simulink model "PID20ejeYanalnivels"  (Simulink 6.6)
settings: Solver=FixedStepDiscrete  StartTime=0.0  StopTime=.002  FixedStep=0.001  RelTol=1e-3
libraries: dsPICdrivers x10, simulink x3
settings Model: Creator=123  LastModifiedBy=123  ProdHWDeviceType=16-bit Generic
settings OptimizationCC: OptimizeModelRefInitCode=on  LifeSpan=1
settings HardwareCC: ProdBitPerInt=16  ProdEndianess=LittleEndian  ProdWordSize=16  ProdHWDeviceType=16-bit Generic  TargetHWDeviceType=32-bit Generic
settings RTWCC: SystemTargetFile=dspic.tlc  TemplateMakefile=dspic_pic30_gcc.tmf  PostCodeGenCommand=dsPIC_Compile()  Description=Embedded Target for Microchip dsPIC (real-time)  ProcessScript=dspic_make_rtw_hook  CustomSource=myQEI.c
settings CodeAppCC: IgnoreCustomStorageClasses=off
settings STFCustomTargetCC: TargetFcnLib=ansi_tfl_tmw.mat  GenFloatMathFcnCalls=ANSI_C  ModelReferenceCompliant=off  IncludeMdlTerminateFcn=off  CombineOutputUpdateFcns=on  SuppressErrorStatus=on  ERTCustomFileBanners=on  SupportContinuousTime=off  SupportNonInlinedSFcns=off  SystemTargetFile=dspic.tlc
settings ERTTargetCC: TargetFcnLib=ansi_tfl_tmw.mat  GenFloatMathFcnCalls=ANSI_C  ModelReferenceCompliant=off  IncludeMdlTerminateFcn=off  SuppressErrorStatus=on  ModelStepFunctionPrototypeControlCompliant=off  InlinedParameterPlacement=NonHierarchical  ERTSrcFileBannerTemplate=dsPIC_code_template.cgt  ERTHdrFileBannerTemplate=dsPIC_code_template.cgt  ERTDataSrcFileTemplate=dsPIC_code_template.cgt  ERTDataHdrFileTemplate=dsPIC_code_template.cgt  ERTCustomFileTemplate=dsPIC_main.tlc
settings CustomProperty: DataType=string  Value=C:\PROGRA~2\MATLAB\R2007a\rtw\bin\win32\gmake

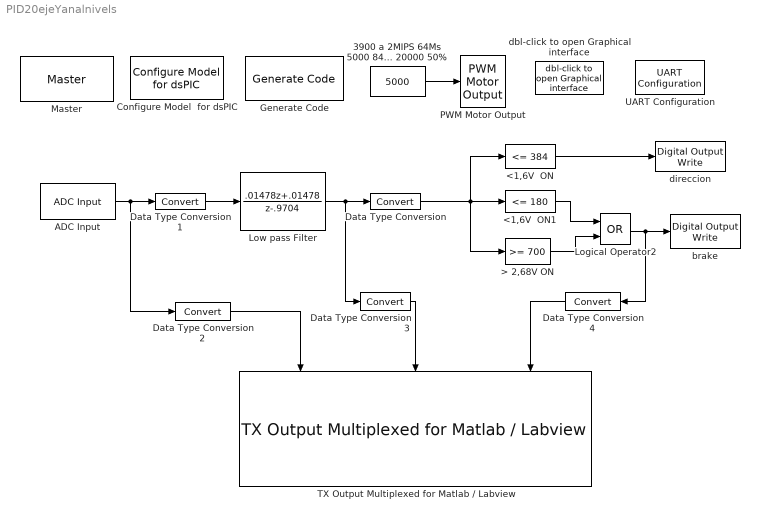
== system PID20ejeYanalnivels ==
  3900 a 2MIPS 64Ms 5000 84Ms 40000 full 20000 50% : Constant  Value=5000  OutDataTypeMode=uint16  SampleTime=.001
  <1,6V  ON : simulink/Logic and Bit Operations/Compare To Constant  SystemSampleTime=-1  relop=<=  const=384  LogicOutDataTypeMode=boolean  ZeroCross=off
  <1,6V  ON1 : simulink/Logic and Bit Operations/Compare To Constant  SystemSampleTime=-1  relop=<=  const=180  LogicOutDataTypeMode=boolean  ZeroCross=off
  > 2,68V ON : simulink/Logic and Bit Operations/Compare To Constant  SystemSampleTime=-1  relop=>=  const=700  LogicOutDataTypeMode=boolean  ZeroCross=off
  ADC Input : dsPICdrivers/Peripheral I//O/ADC Input  Tag=dsPIC_ADC  Priority=5  ADC_TYPE=10 bits  ADC_MODE=Continuous sampling & get last channel value  NbrSampleStep=1  VoltRefpopup="AVdd  -  AVss"  OutFormatBitspopup=0000 00dd dddd dddd : Integer  InterruptPriority=1  ANCHANNELS=[0]  MaxName=ANmax = 1024  Rin=1e2  ADCS=9  SAMC=1  Temperature=25  DMAChannel=0  SampleTime=.001  Status="OK  |  Tsmp=1.667e-007 |  T/Channel=2.167e-006 |  Tall=2.167e-006"
  Configure Model  for dsPIC : dsPICdrivers/Simulink Configuration/Configure Model  for dsPIC
  Data Type Conversion : DataTypeConversion  OutDataTypeMode=uint16  SampleTime=.001
  Data Type Conversion1 : DataTypeConversion  OutDataTypeMode=double  SampleTime=.001
  Data Type Conversion2 : DataTypeConversion  OutDataTypeMode=int16  SampleTime=.001
  Data Type Conversion3 : DataTypeConversion  OutDataTypeMode=int16  SampleTime=.001
  Data Type Conversion4 : DataTypeConversion  Orientation=left  OutDataTypeMode=int16  SampleTime=.001
  Generate Code : dsPICdrivers/Simulink Configuration/Generate Code
  Logical Operator2 : Logic  Operator=OR  AllPortsSameDT=off  OutDataTypeMode=Boolean  SampleTime=.001
  Low pass Filter : DiscreteTransferFcn  Numerator="[.01478  .01478]"  Denominator=[1 -.9704]  SampleTime=.001
  Master : dsPICdrivers/Master  Tag=dsPIC_MASTER  Priority=1  TimeStepType=Timer1  picType=30f4012  fcy=30e6  Quartz_33f=5e6  PLLActive_33f=off  fcyDesired_33f=0  tmr1="[1  29999  0]"  tmr1Info="Time Step : 0.001  ;   Error : 0%  PR1=29999"  tmr2345="[0  0  0  0]"  tmr2345cfg=[-1 -1 -1 -1]  IOautoConf=on  typePort="[ 0   0   0   0   0   0   0   0   0   0   0   0   0   0   0   0   8   0   0   0   0   0   0   0   0   0   0   0   0   0   0   0   0   0   0   0   0   0   0   0   0   0   0   0   0   0   0   0  10  10   0   0   0   0   0   0   0   0   0   0   0   0   0   0  11   0   0   0   0   0   0   0   0   0   0   0   0   0   0   0   0   0   4   5   0   0   0   0   0   0   0   0   0   0   0   0   0   0   0   0   0   0   0   0   0   0   0   0   0   0   0   0 ]"  TRIS="[ 65535  65535  65535  65532  65535  65535  65535 ]"  ADPCFG=0  MasterBusyPort=None  MasterOverloadPort=None  FOSC=FRC_PLL16  ClockSwitchMonitor=Both disabled  TempProtection_33f=TEMP_ON  FPBOR=PBOR_OFF  PWRT=PWRT_OFF  MCLR=MCLR_DIS  PowerSave=off  OverrideFcy=off  NewFcy=1e6
  PWM Motor Output : dsPICdrivers/Peripheral I//O/PWM Motor Output  Tag=dsPIC_PWM_Motor  Priority=5  InputEnableChk=off  InputPeriodeChk=off  Channel=[1 ]  TPeriode=.01  PrescalerValue=16  PeriodeInteger=18750  MaxName='PWM'  Centered=off  HChannelON=off  Info="Nbr Bits : 15.1946  ||  PWM = 37500  ||  Prescaler = 16"  Delay=0  IntPriority=5  nbrPwmChannelPIC=3  Status=OK
  TX Output Multiplexed for Matlab / Labview : dsPICdrivers/Serial PORT/TX Output Multiplexed for Matlab // Labview  Tag=dsPIC_TX_Multiplexed  Orientation=down  Priority=5  UART=1  CleverSpreadingChk=on  CleverSpreading=1  CHANNEL=[0 1 2 ]  CHANNELBLOCKED=[]  CHANNELBLOCKED_BITEWISE=0  Status=OK
  UART Configuration : dsPICdrivers/Serial PORT/UART Configuration  Tag=dsPIC_config_UART  Priority=2  UART=1  proposed_BAUD=115200  ALT_TX_RX=off  InterruptTxWhen=When Transmit Buffer is empty  TXInterruptPri=1  TxBufferSize=32  TXEN=on  InterruptRxWhen=When Receive Buffer is full (contain 4 characters)  RXInterruptPri=2  RxBufferSize=32  BAUD=115200  UxBRG=15  Info="UxBRG = 15   ||  Real Baud : 117188   ||  % error : 1.7253  ||  max 11.7188 Bytes / Step"  RealBaud=0
  brake : dsPICdrivers/Digital I//O/Digital Output Write  Tag=dsPIC_Digital_Output  Priority=5  PORT=D  Pin=[1]  Simultaneous=off  OrderingInOutPopup=None
  dbl-click to open Graphical interface : dsPICdrivers/Serial PORT/dbl-click to open Graphical interface  SystemSampleTime=-1  Nothing=0
  direccion : dsPICdrivers/Digital I//O/Digital Output Write  Tag=dsPIC_Digital_Output  Priority=5  PORT=D  Pin=[0]  Simultaneous=off  OrderingInOutPopup=None
  wires:
  Low pass Filter/1 -> Data Type Conversion/1, Data Type Conversion3/1
  Data Type Conversion/1 -> > 2,68V ON/1, <1,6V  ON/1, <1,6V  ON1/1
  Data Type Conversion1/1 -> Low pass Filter/1
  ADC Input/1 -> Data Type Conversion1/1, Data Type Conversion2/1
  <1,6V  ON/1 -> direccion/1
  > 2,68V ON/1 -> Logical Operator2/2
  <1,6V  ON1/1 -> Logical Operator2/1
  Logical Operator2/1 -> brake/1, Data Type Conversion4/1
  3900 a 2MIPS 64Ms 5000 84Ms 40000 full 20000 50%/1 -> PWM Motor Output/1
  Data Type Conversion2/1 -> TX Output Multiplexed for Matlab / Labview/1
  Data Type Conversion3/1 -> TX Output Multiplexed for Matlab / Labview/2
  Data Type Conversion4/1 -> TX Output Multiplexed for Matlab / Labview/3
